simulink library "Model_GridElem_Arc_Fault"  (R2022b)
settings: Solver=VariableStepAuto  StartTime=0.0  StopTime=10.0  RelTol=1e-3
undefined symbols (not defined in the file): DiscIntNeverNeededParam
libraries: powerlib x220, spsVariableResistorLib x3, spsControlledVoltageSourceLib x3, spsGroundLib x1, spsThreePhaseVIMeasurementLib x1
(part 2 of 2)

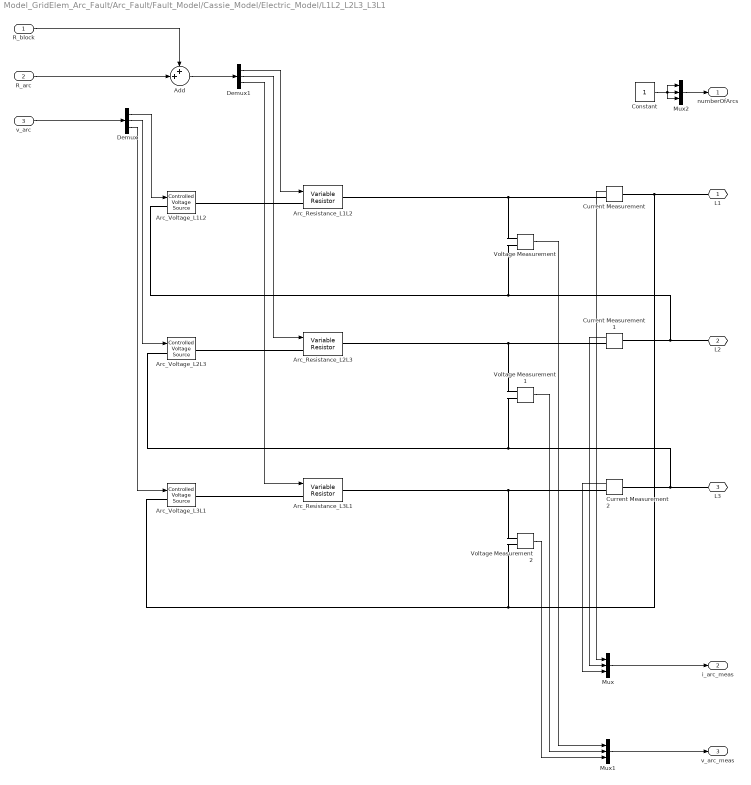
== system Model_GridElem_Arc_Fault/Arc_Fault/Fault_Model/Cassie_Model/Electric_Model/L1L2_L2L3_L3L1 ==
  R_block : Inport
  R_arc : Inport  Port=2
  v_arc : Inport  Port=3
  Add : Sum  Inputs=++|
  Arc_Resistance_L1L2 : powerlib/Elements/Variable Resistor  Rabsmin=1e-6
  Arc_Resistance_L2L3 : powerlib/Elements/Variable Resistor  Rabsmin=1e-6
  Arc_Resistance_L3L1 : powerlib/Elements/Variable Resistor  Rabsmin=1e-6
  Arc_Voltage_L1L2 : powerlib/Electrical Sources/Controlled Voltage Source  Initialize=on  Source_Type=AC  Amplitude=0  Phase=0  Frequency=0  Measurements=None
  Arc_Voltage_L2L3 : powerlib/Electrical Sources/Controlled Voltage Source  Initialize=on  Source_Type=AC  Amplitude=0  Phase=0  Frequency=0  Measurements=None
  Arc_Voltage_L3L1 : powerlib/Electrical Sources/Controlled Voltage Source  Initialize=on  Source_Type=AC  Amplitude=0  Phase=0  Frequency=0  Measurements=None
  Constant : Constant
  Current Measurement : powerlib/Measurements/Current Measurement  PhasorSimulation=off  OutputType=Complex  PSBequivalent=0
  Current Measurement1 : powerlib/Measurements/Current Measurement  PhasorSimulation=off  OutputType=Complex  PSBequivalent=0
  Current Measurement2 : powerlib/Measurements/Current Measurement  PhasorSimulation=off  OutputType=Complex  PSBequivalent=0
  Demux : Demux  Outputs=3
  Demux1 : Demux  Outputs=3
  Mux : Mux  Inputs=3
  Mux1 : Mux  Inputs=3
  Mux2 : Mux  Inputs=3
  Voltage Measurement : powerlib/Measurements/Voltage Measurement  PhasorSimulation=off  OutputType=Complex  PSBequivalent=0
  Voltage Measurement1 : powerlib/Measurements/Voltage Measurement  PhasorSimulation=off  OutputType=Complex  PSBequivalent=0
  Voltage Measurement2 : powerlib/Measurements/Voltage Measurement  PhasorSimulation=off  OutputType=Complex  PSBequivalent=0
  L1 : PMIOPort  Side=Right
  L2 : PMIOPort  Port=2  Side=Right
  L3 : PMIOPort  Port=3  Side=Right
  numberOfArcs : Outport
  i_arc_meas : Outport  Port=2
  v_arc_meas : Outport  Port=3
  wires:
  Constant/1 -> Mux2/2, Mux2/1, Mux2/3
  Mux2/1 -> numberOfArcs/1
  R_arc/1 -> Add/2
  Add/1 -> Demux1/1
  Voltage Measurement2/1 -> Mux1/3
  Voltage Measurement1/1 -> Mux1/2
  Voltage Measurement/1 -> Mux1/1
  Current Measurement2/1 -> Mux/3
  Current Measurement1/1 -> Mux/2
  Current Measurement/1 -> Mux/1
  Mux1/1 -> v_arc_meas/1
  Mux/1 -> i_arc_meas/1
  Demux/2 -> Arc_Voltage_L2L3/1
  Demux1/2 -> Arc_Resistance_L2L3/1
  Demux/3 -> Arc_Voltage_L3L1/1
  Demux1/1 -> Arc_Resistance_L1L2/1
  v_arc/1 -> Demux/1
  Demux/1 -> Arc_Voltage_L1L2/1
  Demux1/3 -> Arc_Resistance_L3L1/1
  R_block/1 -> Add/1
  connections:
  Arc_Resistance_L3L1/RConn1 -- Voltage Measurement2/LConn1 -- Current Measurement2/RConn1
  Arc_Resistance_L2L3/RConn1 -- Voltage Measurement1/LConn1 -- Current Measurement1/RConn1
  Voltage Measurement/LConn1 -- Arc_Resistance_L1L2/RConn1 -- Current Measurement/RConn1
  Current Measurement1/LConn1 -- Voltage Measurement/LConn2 -- Arc_Voltage_L1L2/LConn1 -- L2/RConn1
  L3/RConn1 -- Current Measurement2/LConn1 -- Voltage Measurement1/LConn2 -- Arc_Voltage_L2L3/LConn1
  Current Measurement/LConn1 -- L1/RConn1 -- Voltage Measurement2/LConn2 -- Arc_Voltage_L3L1/LConn1
  Arc_Voltage_L2L3/RConn1 -- Arc_Resistance_L2L3/LConn1
  Arc_Voltage_L3L1/RConn1 -- Arc_Resistance_L3L1/LConn1
  Arc_Voltage_L1L2/RConn1 -- Arc_Resistance_L1L2/LConn1

== system Model_GridElem_Arc_Fault/Arc_Fault/Fault_Model/Mayr_Model/Electric_Model/L1G ==
  R_block : Inport
  R_arc : Inport  Port=2
  v_arc : Inport  Port=3
  Add : Sum  Inputs=++|
  Arc_Resistance_L1G : powerlib/Elements/Variable Resistor  Rabsmin=1e-6
  Arc_Voltage_L1G : powerlib/Electrical Sources/Controlled Voltage Source  Initialize=on  Source_Type=AC  Amplitude=0  Phase=0  Frequency=0  Measurements=None
  Constant : Constant
  Current Measurement : powerlib/Measurements/Current Measurement  PhasorSimulation=off  OutputType=Complex  PSBequivalent=0
  Ground{,1..3} (4 alike) : powerlib/Elements/Ground  LConnTagsString=a
  Terminator : Terminator
  Terminator1 : Terminator
  Voltage Measurement : powerlib/Measurements/Voltage Measurement  PhasorSimulation=off  OutputType=Complex  PSBequivalent=0
  Voltage Measurement1 : powerlib/Measurements/Voltage Measurement  PhasorSimulation=off  OutputType=Complex  PSBequivalent=0
  Voltage Measurement2 : powerlib/Measurements/Voltage Measurement  PhasorSimulation=off  OutputType=Complex  PSBequivalent=0
  L1 : PMIOPort  Side=Right
  L2 : PMIOPort  Port=2  Side=Right
  L3 : PMIOPort  Port=3  Side=Right
  numberOfArcs : Outport
  i_arc_meas : Outport  Port=2
  v_arc_meas : Outport  Port=3
  wires:
  Constant/1 -> numberOfArcs/1
  Add/1 -> Arc_Resistance_L1G/1
  R_block/1 -> Add/1
  R_arc/1 -> Add/2
  Voltage Measurement1/1 -> Terminator1/1
  Current Measurement/1 -> i_arc_meas/1
  v_arc/1 -> Arc_Voltage_L1G/1
  Voltage Measurement2/1 -> Terminator/1
  Voltage Measurement/1 -> v_arc_meas/1
  connections:
  Voltage Measurement1/LConn2 -- Ground2/LConn1
  Voltage Measurement1/LConn1 -- L2/RConn1
  Arc_Voltage_L1G/RConn1 -- Arc_Resistance_L1G/LConn1
  Voltage Measurement2/LConn2 -- Ground3/LConn1
  Ground1/LConn1 -- Voltage Measurement/LConn2
  Voltage Measurement2/LConn1 -- L3/RConn1
  Current Measurement/LConn1 -- L1/RConn1
  Ground/LConn1 -- Arc_Voltage_L1G/LConn1
  Voltage Measurement/LConn1 -- Arc_Resistance_L1G/RConn1 -- Current Measurement/RConn1

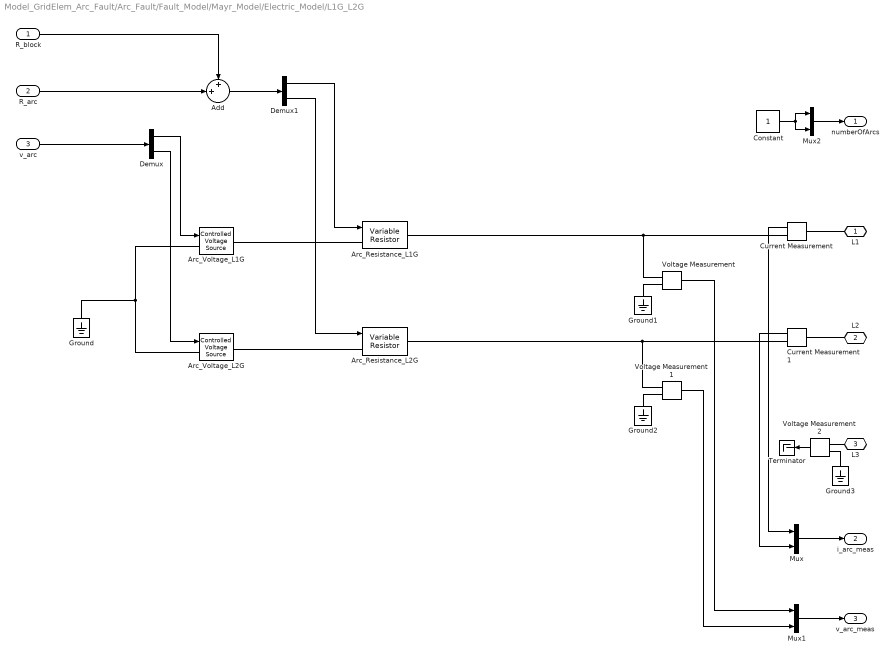
== system Model_GridElem_Arc_Fault/Arc_Fault/Fault_Model/Mayr_Model/Electric_Model/L1G_L2G ==
  R_block : Inport
  R_arc : Inport  Port=2
  v_arc : Inport  Port=3
  Add : Sum  Inputs=++|
  Arc_Resistance_L1G : powerlib/Elements/Variable Resistor  Rabsmin=1e-6
  Arc_Resistance_L2G : powerlib/Elements/Variable Resistor  Rabsmin=1e-6
  Arc_Voltage_L1G : powerlib/Electrical Sources/Controlled Voltage Source  Initialize=on  Source_Type=AC  Amplitude=0  Phase=0  Frequency=0  Measurements=None
  Arc_Voltage_L2G : powerlib/Electrical Sources/Controlled Voltage Source  Initialize=on  Source_Type=AC  Amplitude=0  Phase=0  Frequency=0  Measurements=None
  Constant : Constant
  Current Measurement : powerlib/Measurements/Current Measurement  PhasorSimulation=off  OutputType=Complex  PSBequivalent=0
  Current Measurement1 : powerlib/Measurements/Current Measurement  PhasorSimulation=off  OutputType=Complex  PSBequivalent=0
  Demux : Demux  Outputs=2
  Demux1 : Demux  Outputs=2
  Ground{,1..3} (4 alike) : powerlib/Elements/Ground  LConnTagsString=a
  Mux : Mux  Inputs=2
  Mux1 : Mux  Inputs=2
  Mux2 : Mux  Inputs=2
  Terminator : Terminator
  Voltage Measurement : powerlib/Measurements/Voltage Measurement  PhasorSimulation=off  OutputType=Complex  PSBequivalent=0
  Voltage Measurement1 : powerlib/Measurements/Voltage Measurement  PhasorSimulation=off  OutputType=Complex  PSBequivalent=0
  Voltage Measurement2 : powerlib/Measurements/Voltage Measurement  PhasorSimulation=off  OutputType=Complex  PSBequivalent=0
  L1 : PMIOPort  Side=Right
  L2 : PMIOPort  Port=2  Side=Right
  L3 : PMIOPort  Port=3  Side=Right
  numberOfArcs : Outport
  i_arc_meas : Outport  Port=2
  v_arc_meas : Outport  Port=3
  wires:
  Constant/1 -> Mux2/1, Mux2/2
  Mux2/1 -> numberOfArcs/1
  R_block/1 -> Add/1
  Add/1 -> Demux1/1
  R_arc/1 -> Add/2
  Voltage Measurement2/1 -> Terminator/1
  Voltage Measurement1/1 -> Mux1/2
  Voltage Measurement/1 -> Mux1/1
  Current Measurement1/1 -> Mux/2
  Current Measurement/1 -> Mux/1
  Mux1/1 -> v_arc_meas/1
  Mux/1 -> i_arc_meas/1
  Demux/2 -> Arc_Voltage_L2G/1
  Demux1/2 -> Arc_Resistance_L2G/1
  Demux1/1 -> Arc_Resistance_L1G/1
  v_arc/1 -> Demux/1
  Demux/1 -> Arc_Voltage_L1G/1
  connections:
  Voltage Measurement2/LConn2 -- Ground3/LConn1
  Ground2/LConn1 -- Voltage Measurement1/LConn2
  Ground1/LConn1 -- Voltage Measurement/LConn2
  Current Measurement1/LConn1 -- L2/RConn1
  Voltage Measurement1/LConn1 -- Arc_Resistance_L2G/RConn1 -- Current Measurement1/RConn1
  Current Measurement/LConn1 -- L1/RConn1
  Voltage Measurement/LConn1 -- Arc_Resistance_L1G/RConn1 -- Current Measurement/RConn1
  Arc_Voltage_L1G/RConn1 -- Arc_Resistance_L1G/LConn1
  Arc_Voltage_L2G/RConn1 -- Arc_Resistance_L2G/LConn1
  Voltage Measurement2/LConn1 -- L3/RConn1
  Arc_Voltage_L1G/LConn1 -- Arc_Voltage_L2G/LConn1 -- Ground/LConn1

== system Model_GridElem_Arc_Fault/Arc_Fault/Fault_Model/Mayr_Model/Electric_Model/L1G_L2G_L3G ==
  R_block : Inport
  R_arc : Inport  Port=2
  v_arc : Inport  Port=3
  Add : Sum  Inputs=++|
  Arc_Resistance_L1G : powerlib/Elements/Variable Resistor  Rabsmin=1e-6
  Arc_Resistance_L2G : powerlib/Elements/Variable Resistor  Rabsmin=1e-6
  Arc_Resistance_L3G : powerlib/Elements/Variable Resistor  Rabsmin=1e-6
  Arc_Voltage_L1G : powerlib/Electrical Sources/Controlled Voltage Source  Initialize=on  Source_Type=AC  Amplitude=0  Phase=0  Frequency=0  Measurements=None
  Arc_Voltage_L2G : powerlib/Electrical Sources/Controlled Voltage Source  Initialize=on  Source_Type=AC  Amplitude=0  Phase=0  Frequency=0  Measurements=None
  Arc_Voltage_L3G : powerlib/Electrical Sources/Controlled Voltage Source  Initialize=on  Source_Type=AC  Amplitude=0  Phase=0  Frequency=0  Measurements=None
  Constant : Constant
  Demux : Demux  Outputs=3
  Demux1 : Demux  Outputs=3
  Ground : powerlib/Elements/Ground  LConnTagsString=a
  Mux : Mux  Inputs=3
  Three-Phase V-I Measurement : powerlib/Measurements/Three-Phase V-I Measurement  VoltageMeasurement=phase-to-ground  SetLabelV=off  LabelV=Vabc  Vpu=off  VpuLL=off  CurrentMeasurement=yes  SetLabelI=off  LabelI=Iabc  Ipu=off  Pbase=100e6  Vbase=500e3  OutputType=Complex  PhasorSimulation=off  PSBequivalent=0
  L1 : PMIOPort  Side=Right
  L2 : PMIOPort  Port=2  Side=Right
  L3 : PMIOPort  Port=3  Side=Right
  numberOfArcs : Outport
  i_arc_meas : Outport  Port=2
  v_arc_meas : Outport  Port=3
  wires:
  Constant/1 -> Mux/2, Mux/1, Mux/3
  Mux/1 -> numberOfArcs/1
  R_block/1 -> Add/1
  Add/1 -> Demux1/1
  R_arc/1 -> Add/2
  Demux1/1 -> Arc_Resistance_L1G/1
  Demux1/2 -> Arc_Resistance_L2G/1
  Demux1/3 -> Arc_Resistance_L3G/1
  Demux/1 -> Arc_Voltage_L1G/1
  Demux/2 -> Arc_Voltage_L2G/1
  Demux/3 -> Arc_Voltage_L3G/1
  Three-Phase V-I Measurement/1 -> v_arc_meas/1
  Three-Phase V-I Measurement/2 -> i_arc_meas/1
  v_arc/1 -> Demux/1
  connections:
  Three-Phase V-I Measurement/LConn3 -- L3/RConn1
  Three-Phase V-I Measurement/LConn2 -- L2/RConn1
  Three-Phase V-I Measurement/LConn1 -- L1/RConn1
  Arc_Resistance_L3G/RConn1 -- Three-Phase V-I Measurement/RConn3
  Arc_Resistance_L1G/RConn1 -- Three-Phase V-I Measurement/RConn1
  Ground/LConn1 -- Arc_Voltage_L3G/LConn1 -- Arc_Voltage_L2G/LConn1 -- Arc_Voltage_L1G/LConn1
  Arc_Voltage_L3G/RConn1 -- Arc_Resistance_L3G/LConn1
  Arc_Voltage_L2G/RConn1 -- Arc_Resistance_L2G/LConn1
  Arc_Voltage_L1G/RConn1 -- Arc_Resistance_L1G/LConn1
  Three-Phase V-I Measurement/RConn2 -- Arc_Resistance_L2G/RConn1

== system Model_GridElem_Arc_Fault/Arc_Fault/Fault_Model/Mayr_Model/Electric_Model/L1L2 ==
  R_block : Inport
  R_arc : Inport  Port=2
  v_arc : Inport  Port=3
  Add : Sum  Inputs=++|
  Arc_Resistance_L1L2 : powerlib/Elements/Variable Resistor  Rabsmin=1e-6
  Arc_Voltage_L1L2 : powerlib/Electrical Sources/Controlled Voltage Source  Initialize=on  Source_Type=AC  Amplitude=0  Phase=0  Frequency=0  Measurements=None
  Constant : Constant
  Current Measurement : powerlib/Measurements/Current Measurement  PhasorSimulation=off  OutputType=Complex  PSBequivalent=0
  Ground : powerlib/Elements/Ground  LConnTagsString=a
  Terminator : Terminator
  Voltage Measurement : powerlib/Measurements/Voltage Measurement  PhasorSimulation=off  OutputType=Complex  PSBequivalent=0
  Voltage Measurement1 : powerlib/Measurements/Voltage Measurement  PhasorSimulation=off  OutputType=Complex  PSBequivalent=0
  L1 : PMIOPort  Side=Right
  L2 : PMIOPort  Port=2  Side=Right
  L3 : PMIOPort  Port=3  Side=Right
  numberOfArcs : Outport
  i_arc_meas : Outport  Port=2
  v_arc_meas : Outport  Port=3
  wires:
  Constant/1 -> numberOfArcs/1
  R_block/1 -> Add/1
  Add/1 -> Arc_Resistance_L1L2/1
  R_arc/1 -> Add/2
  Voltage Measurement1/1 -> Terminator/1
  v_arc/1 -> Arc_Voltage_L1L2/1
  Voltage Measurement/1 -> v_arc_meas/1
  Current Measurement/1 -> i_arc_meas/1
  connections:
  Voltage Measurement1/LConn2 -- Ground/LConn1
  Voltage Measurement1/LConn1 -- L3/RConn1
  Arc_Voltage_L1L2/RConn1 -- Arc_Resistance_L1L2/LConn1
  Current Measurement/LConn1 -- L1/RConn1
  L2/RConn1 -- Arc_Voltage_L1L2/LConn1 -- Voltage Measurement/LConn2
  Voltage Measurement/LConn1 -- Arc_Resistance_L1L2/RConn1 -- Current Measurement/RConn1

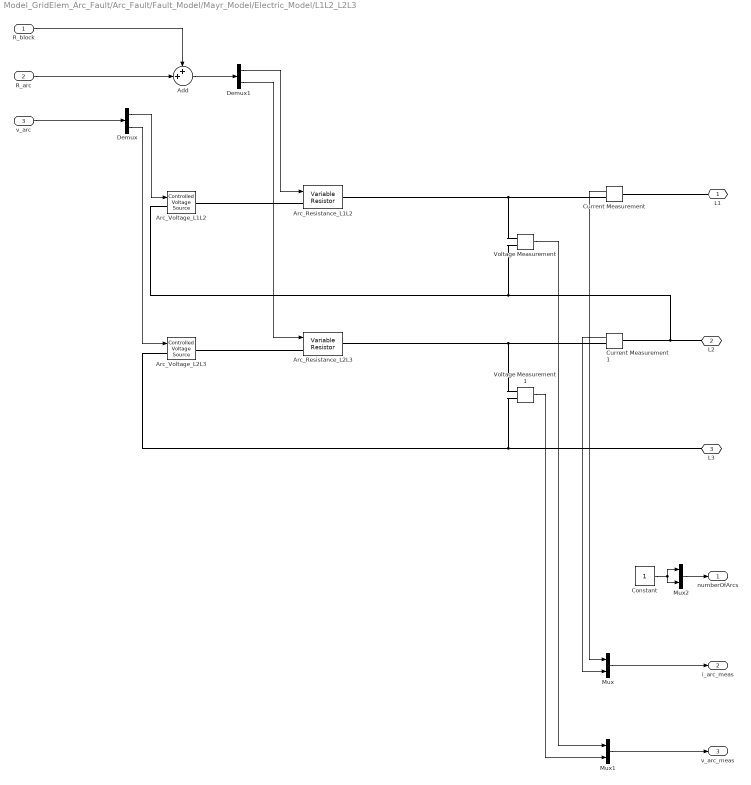
== system Model_GridElem_Arc_Fault/Arc_Fault/Fault_Model/Mayr_Model/Electric_Model/L1L2_L2L3 ==
  R_block : Inport
  R_arc : Inport  Port=2
  v_arc : Inport  Port=3
  Add : Sum  Inputs=++|
  Arc_Resistance_L1L2 : powerlib/Elements/Variable Resistor  Rabsmin=1e-6
  Arc_Resistance_L2L3 : powerlib/Elements/Variable Resistor  Rabsmin=1e-6
  Arc_Voltage_L1L2 : powerlib/Electrical Sources/Controlled Voltage Source  Initialize=on  Source_Type=AC  Amplitude=0  Phase=0  Frequency=0  Measurements=None
  Arc_Voltage_L2L3 : powerlib/Electrical Sources/Controlled Voltage Source  Initialize=on  Source_Type=AC  Amplitude=0  Phase=0  Frequency=0  Measurements=None
  Constant : Constant
  Current Measurement : powerlib/Measurements/Current Measurement  PhasorSimulation=off  OutputType=Complex  PSBequivalent=0
  Current Measurement1 : powerlib/Measurements/Current Measurement  PhasorSimulation=off  OutputType=Complex  PSBequivalent=0
  Demux : Demux  Outputs=2
  Demux1 : Demux  Outputs=2
  Mux : Mux  Inputs=2
  Mux1 : Mux  Inputs=2
  Mux2 : Mux  Inputs=2
  Voltage Measurement : powerlib/Measurements/Voltage Measurement  PhasorSimulation=off  OutputType=Complex  PSBequivalent=0
  Voltage Measurement1 : powerlib/Measurements/Voltage Measurement  PhasorSimulation=off  OutputType=Complex  PSBequivalent=0
  L1 : PMIOPort  Side=Right
  L2 : PMIOPort  Port=2  Side=Right
  L3 : PMIOPort  Port=3  Side=Right
  numberOfArcs : Outport
  i_arc_meas : Outport  Port=2
  v_arc_meas : Outport  Port=3
  wires:
  Constant/1 -> Mux2/1, Mux2/2
  Mux2/1 -> numberOfArcs/1
  R_block/1 -> Add/1
  R_arc/1 -> Add/2
  Add/1 -> Demux1/1
  Demux1/2 -> Arc_Resistance_L2L3/1
  Voltage Measurement1/1 -> Mux1/2
  Voltage Measurement/1 -> Mux1/1
  Demux/2 -> Arc_Voltage_L2L3/1
  Demux1/1 -> Arc_Resistance_L1L2/1
  Mux1/1 -> v_arc_meas/1
  Demux/1 -> Arc_Voltage_L1L2/1
  v_arc/1 -> Demux/1
  Current Measurement1/1 -> Mux/2
  Mux/1 -> i_arc_meas/1
  Current Measurement/1 -> Mux/1
  connections:
  Arc_Voltage_L1L2/RConn1 -- Arc_Resistance_L1L2/LConn1
  Arc_Voltage_L2L3/RConn1 -- Arc_Resistance_L2L3/LConn1
  Voltage Measurement1/LConn1 -- Arc_Resistance_L2L3/RConn1 -- Current Measurement1/RConn1
  Arc_Voltage_L1L2/LConn1 -- L2/RConn1 -- Current Measurement1/LConn1 -- Voltage Measurement/LConn2
  L3/RConn1 -- Arc_Voltage_L2L3/LConn1 -- Voltage Measurement1/LConn2
  Voltage Measurement/LConn1 -- Arc_Resistance_L1L2/RConn1 -- Current Measurement/RConn1
  Current Measurement/LConn1 -- L1/RConn1

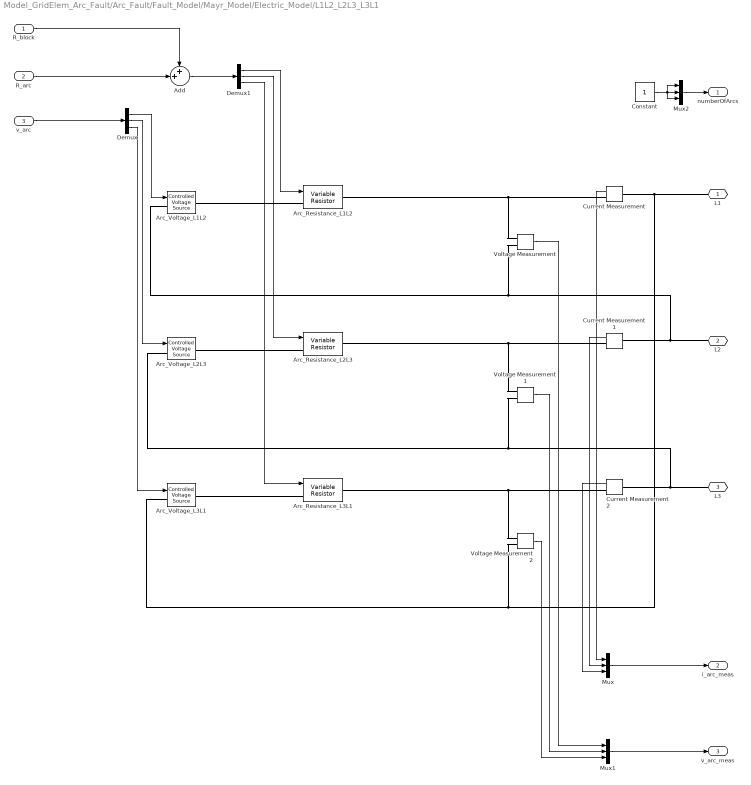
== system Model_GridElem_Arc_Fault/Arc_Fault/Fault_Model/Mayr_Model/Electric_Model/L1L2_L2L3_L3L1 ==
  R_block : Inport
  R_arc : Inport  Port=2
  v_arc : Inport  Port=3
  Add : Sum  Inputs=++|
  Arc_Resistance_L1L2 : powerlib/Elements/Variable Resistor  Rabsmin=1e-6
  Arc_Resistance_L2L3 : powerlib/Elements/Variable Resistor  Rabsmin=1e-6
  Arc_Resistance_L3L1 : powerlib/Elements/Variable Resistor  Rabsmin=1e-6
  Arc_Voltage_L1L2 : powerlib/Electrical Sources/Controlled Voltage Source  Initialize=on  Source_Type=AC  Amplitude=0  Phase=0  Frequency=0  Measurements=None
  Arc_Voltage_L2L3 : powerlib/Electrical Sources/Controlled Voltage Source  Initialize=on  Source_Type=AC  Amplitude=0  Phase=0  Frequency=0  Measurements=None
  Arc_Voltage_L3L1 : powerlib/Electrical Sources/Controlled Voltage Source  Initialize=on  Source_Type=AC  Amplitude=0  Phase=0  Frequency=0  Measurements=None
  Constant : Constant
  Current Measurement : powerlib/Measurements/Current Measurement  PhasorSimulation=off  OutputType=Complex  PSBequivalent=0
  Current Measurement1 : powerlib/Measurements/Current Measurement  PhasorSimulation=off  OutputType=Complex  PSBequivalent=0
  Current Measurement2 : powerlib/Measurements/Current Measurement  PhasorSimulation=off  OutputType=Complex  PSBequivalent=0
  Demux : Demux  Outputs=3
  Demux1 : Demux  Outputs=3
  Mux : Mux  Inputs=3
  Mux1 : Mux  Inputs=3
  Mux2 : Mux  Inputs=3
  Voltage Measurement : powerlib/Measurements/Voltage Measurement  PhasorSimulation=off  OutputType=Complex  PSBequivalent=0
  Voltage Measurement1 : powerlib/Measurements/Voltage Measurement  PhasorSimulation=off  OutputType=Complex  PSBequivalent=0
  Voltage Measurement2 : powerlib/Measurements/Voltage Measurement  PhasorSimulation=off  OutputType=Complex  PSBequivalent=0
  L1 : PMIOPort  Side=Right
  L2 : PMIOPort  Port=2  Side=Right
  L3 : PMIOPort  Port=3  Side=Right
  numberOfArcs : Outport
  i_arc_meas : Outport  Port=2
  v_arc_meas : Outport  Port=3
  wires:
  Constant/1 -> Mux2/2, Mux2/1, Mux2/3
  Mux2/1 -> numberOfArcs/1
  R_arc/1 -> Add/2
  Add/1 -> Demux1/1
  Voltage Measurement2/1 -> Mux1/3
  Voltage Measurement1/1 -> Mux1/2
  Voltage Measurement/1 -> Mux1/1
  Current Measurement2/1 -> Mux/3
  Current Measurement1/1 -> Mux/2
  Current Measurement/1 -> Mux/1
  Mux1/1 -> v_arc_meas/1
  Mux/1 -> i_arc_meas/1
  Demux/2 -> Arc_Voltage_L2L3/1
  Demux1/2 -> Arc_Resistance_L2L3/1
  Demux/3 -> Arc_Voltage_L3L1/1
  Demux1/1 -> Arc_Resistance_L1L2/1
  v_arc/1 -> Demux/1
  Demux/1 -> Arc_Voltage_L1L2/1
  Demux1/3 -> Arc_Resistance_L3L1/1
  R_block/1 -> Add/1
  connections:
  Arc_Resistance_L3L1/RConn1 -- Voltage Measurement2/LConn1 -- Current Measurement2/RConn1
  Arc_Resistance_L2L3/RConn1 -- Voltage Measurement1/LConn1 -- Current Measurement1/RConn1
  Voltage Measurement/LConn1 -- Arc_Resistance_L1L2/RConn1 -- Current Measurement/RConn1
  Current Measurement1/LConn1 -- Voltage Measurement/LConn2 -- Arc_Voltage_L1L2/LConn1 -- L2/RConn1
  L3/RConn1 -- Current Measurement2/LConn1 -- Voltage Measurement1/LConn2 -- Arc_Voltage_L2L3/LConn1
  Current Measurement/LConn1 -- L1/RConn1 -- Voltage Measurement2/LConn2 -- Arc_Voltage_L3L1/LConn1
  Arc_Voltage_L2L3/RConn1 -- Arc_Resistance_L2L3/LConn1
  Arc_Voltage_L3L1/RConn1 -- Arc_Resistance_L3L1/LConn1
  Arc_Voltage_L1L2/RConn1 -- Arc_Resistance_L1L2/LConn1

== system Model_GridElem_Arc_Fault/Arc_Fault/Fault_Model/Mayr_Model/Mayr_Arc_Model/Arc_Equations ==
  enable : Inport
  numberOfArcs : Inport  Port=2
  i_abc : Inport  Port=3
  Enable : EnablePort
  1/P : Gain  Gain=1/Mayr_P_0
  1/T : Gain  Gain=1/Mayr_T
  Add : Sum  Inputs=|+-
  Constant : Constant  Value=(Mayr_G_max-Mayr_G_min)/2
  Discrete-Time Integrator : DiscreteIntegrator  ExternalReset=rising  InitialConditionSource=external  SampleTime=-1  LimitOutput=on  UpperSaturationLimit=Mayr_G_max  LowerSaturationLimit=Mayr_G_min  IgnoreLimit=on  ICPrevOutput=DiscIntNeverNeededParam  ICPrevScaledInput=DiscIntNeverNeededParam
  Divide : Product  Inputs=**
  Math Function : Math  Operator=square
  Math Function1 : Math  Operator=reciprocal
  R_arc : Outport
  wires:
  Math Function1/1 -> R_arc/1
  i_abc/1 -> Math Function/1
  Math Function/1 -> 1/P/1
  1/P/1 -> Add/1
  Add/1 -> 1/T/1
  1/T/1 -> Discrete-Time Integrator/1
  enable/1 -> Discrete-Time Integrator/2
  Discrete-Time Integrator/1 -> Math Function1/1, Add/2
  Divide/1 -> Discrete-Time Integrator/3
  Constant/1 -> Divide/1
  numberOfArcs/1 -> Divide/2

== system Model_GridElem_Arc_Fault/Arc_Fault/Fault_Model/Resistor/Electric_Model/L1G ==
  R_block : Inport
  R_arc : Inport  Port=2
  v_arc : Inport  Port=3
  Add : Sum  Inputs=++|
  Arc_Resistance_L1G : powerlib/Elements/Variable Resistor  Rabsmin=1e-6
  Arc_Voltage_L1G : powerlib/Electrical Sources/Controlled Voltage Source  Initialize=on  Source_Type=AC  Amplitude=0  Phase=0  Frequency=0  Measurements=None
  Constant : Constant
  Current Measurement : powerlib/Measurements/Current Measurement  PhasorSimulation=off  OutputType=Complex  PSBequivalent=0
  Ground{,1..3} (4 alike) : powerlib/Elements/Ground  LConnTagsString=a
  Terminator : Terminator
  Terminator1 : Terminator
  Voltage Measurement : powerlib/Measurements/Voltage Measurement  PhasorSimulation=off  OutputType=Complex  PSBequivalent=0
  Voltage Measurement1 : powerlib/Measurements/Voltage Measurement  PhasorSimulation=off  OutputType=Complex  PSBequivalent=0
  Voltage Measurement2 : powerlib/Measurements/Voltage Measurement  PhasorSimulation=off  OutputType=Complex  PSBequivalent=0
  L1 : PMIOPort  Side=Right
  L2 : PMIOPort  Port=2  Side=Right
  L3 : PMIOPort  Port=3  Side=Right
  numberOfArcs : Outport
  i_arc_meas : Outport  Port=2
  v_arc_meas : Outport  Port=3
  wires:
  Voltage Measurement/1 -> v_arc_meas/1
  Voltage Measurement2/1 -> Terminator/1
  v_arc/1 -> Arc_Voltage_L1G/1
  Current Measurement/1 -> i_arc_meas/1
  Voltage Measurement1/1 -> Terminator1/1
  R_arc/1 -> Add/2
  R_block/1 -> Add/1
  Add/1 -> Arc_Resistance_L1G/1
  Constant/1 -> numberOfArcs/1
  connections:
  Current Measurement/RConn1 -- Arc_Resistance_L1G/RConn1 -- Voltage Measurement/LConn1
  Ground/LConn1 -- Arc_Voltage_L1G/LConn1
  Current Measurement/LConn1 -- L1/RConn1
  Voltage Measurement2/LConn1 -- L3/RConn1
  Ground1/LConn1 -- Voltage Measurement/LConn2
  Voltage Measurement2/LConn2 -- Ground3/LConn1
  Arc_Voltage_L1G/RConn1 -- Arc_Resistance_L1G/LConn1
  Voltage Measurement1/LConn1 -- L2/RConn1
  Voltage Measurement1/LConn2 -- Ground2/LConn1

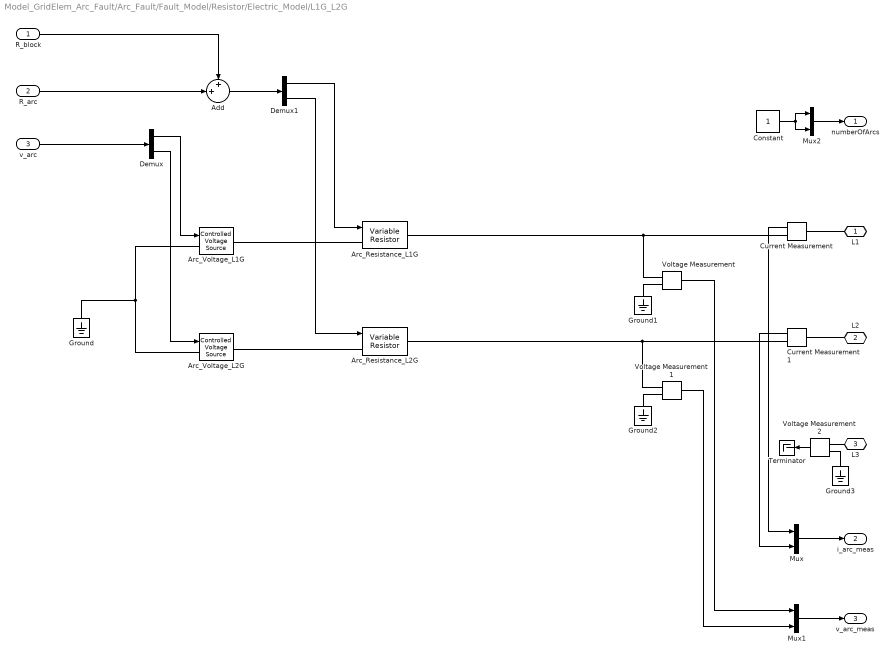
== system Model_GridElem_Arc_Fault/Arc_Fault/Fault_Model/Resistor/Electric_Model/L1G_L2G ==
  R_block : Inport
  R_arc : Inport  Port=2
  v_arc : Inport  Port=3
  Add : Sum  Inputs=++|
  Arc_Resistance_L1G : powerlib/Elements/Variable Resistor  Rabsmin=1e-6
  Arc_Resistance_L2G : powerlib/Elements/Variable Resistor  Rabsmin=1e-6
  Arc_Voltage_L1G : powerlib/Electrical Sources/Controlled Voltage Source  Initialize=on  Source_Type=AC  Amplitude=0  Phase=0  Frequency=0  Measurements=None
  Arc_Voltage_L2G : powerlib/Electrical Sources/Controlled Voltage Source  Initialize=on  Source_Type=AC  Amplitude=0  Phase=0  Frequency=0  Measurements=None
  Constant : Constant
  Current Measurement : powerlib/Measurements/Current Measurement  PhasorSimulation=off  OutputType=Complex  PSBequivalent=0
  Current Measurement1 : powerlib/Measurements/Current Measurement  PhasorSimulation=off  OutputType=Complex  PSBequivalent=0
  Demux : Demux  Outputs=2
  Demux1 : Demux  Outputs=2
  Ground{,1..3} (4 alike) : powerlib/Elements/Ground  LConnTagsString=a
  Mux : Mux  Inputs=2
  Mux1 : Mux  Inputs=2
  Mux2 : Mux  Inputs=2
  Terminator : Terminator
  Voltage Measurement : powerlib/Measurements/Voltage Measurement  PhasorSimulation=off  OutputType=Complex  PSBequivalent=0
  Voltage Measurement1 : powerlib/Measurements/Voltage Measurement  PhasorSimulation=off  OutputType=Complex  PSBequivalent=0
  Voltage Measurement2 : powerlib/Measurements/Voltage Measurement  PhasorSimulation=off  OutputType=Complex  PSBequivalent=0
  L1 : PMIOPort  Side=Right
  L2 : PMIOPort  Port=2  Side=Right
  L3 : PMIOPort  Port=3  Side=Right
  numberOfArcs : Outport
  i_arc_meas : Outport  Port=2
  v_arc_meas : Outport  Port=3
  wires:
  Demux/1 -> Arc_Voltage_L1G/1
  v_arc/1 -> Demux/1
  Demux1/1 -> Arc_Resistance_L1G/1
  Demux1/2 -> Arc_Resistance_L2G/1
  Demux/2 -> Arc_Voltage_L2G/1
  Mux/1 -> i_arc_meas/1
  Mux1/1 -> v_arc_meas/1
  Current Measurement/1 -> Mux/1
  Current Measurement1/1 -> Mux/2
  Voltage Measurement/1 -> Mux1/1
  Voltage Measurement1/1 -> Mux1/2
  Voltage Measurement2/1 -> Terminator/1
  R_arc/1 -> Add/2
  Add/1 -> Demux1/1
  R_block/1 -> Add/1
  Mux2/1 -> numberOfArcs/1
  Constant/1 -> Mux2/2, Mux2/1
  connections:
  Ground/LConn1 -- Arc_Voltage_L2G/LConn1 -- Arc_Voltage_L1G/LConn1
  Voltage Measurement2/LConn1 -- L3/RConn1
  Arc_Voltage_L2G/RConn1 -- Arc_Resistance_L2G/LConn1
  Arc_Voltage_L1G/RConn1 -- Arc_Resistance_L1G/LConn1
  Current Measurement/RConn1 -- Arc_Resistance_L1G/RConn1 -- Voltage Measurement/LConn1
  Current Measurement/LConn1 -- L1/RConn1
  Current Measurement1/RConn1 -- Arc_Resistance_L2G/RConn1 -- Voltage Measurement1/LConn1
  Current Measurement1/LConn1 -- L2/RConn1
  Ground1/LConn1 -- Voltage Measurement/LConn2
  Ground2/LConn1 -- Voltage Measurement1/LConn2
  Voltage Measurement2/LConn2 -- Ground3/LConn1

== system Model_GridElem_Arc_Fault/Arc_Fault/Fault_Model/Resistor/Electric_Model/L1G_L2G_L3G ==
  R_block : Inport
  R_arc : Inport  Port=2
  v_arc : Inport  Port=3
  Add : Sum  Inputs=++|
  Arc_Resistance_L1G : spsVariableResistorLib/Variable Resistor  Rabsmin=1e-6
  Arc_Resistance_L2G : spsVariableResistorLib/Variable Resistor  Rabsmin=1e-6
  Arc_Resistance_L3G : spsVariableResistorLib/Variable Resistor  Rabsmin=1e-6
  Arc_Voltage_L1G : spsControlledVoltageSourceLib/Controlled Voltage Source  Initialize=on  Source_Type=AC  Amplitude=0  Phase=0  Frequency=0  Measurements=None
  Arc_Voltage_L2G : spsControlledVoltageSourceLib/Controlled Voltage Source  Initialize=on  Source_Type=AC  Amplitude=0  Phase=0  Frequency=0  Measurements=None
  Arc_Voltage_L3G : spsControlledVoltageSourceLib/Controlled Voltage Source  Initialize=on  Source_Type=AC  Amplitude=0  Phase=0  Frequency=0  Measurements=None
  Constant : Constant
  Demux : Demux  Outputs=3
  Demux1 : Demux  Outputs=3
  Ground : spsGroundLib/Ground  LConnTagsString=a
  Mux : Mux  Inputs=3
  Three-Phase V-I Measurement : spsThreePhaseVIMeasurementLib/Three-Phase V-I Measurement  VoltageMeasurement=phase-to-ground  SetLabelV=off  LabelV=Vabc  Vpu=off  VpuLL=off  CurrentMeasurement=yes  SetLabelI=off  LabelI=Iabc  Ipu=off  Pbase=100e6  Vbase=500e3  OutputType=Complex  PhasorSimulation=off  PSBequivalent=0
  L1 : PMIOPort  Side=Right
  L2 : PMIOPort  Port=2  Side=Right
  L3 : PMIOPort  Port=3  Side=Right
  numberOfArcs : Outport
  i_arc_meas : Outport  Port=2
  v_arc_meas : Outport  Port=3
  wires:
  v_arc/1 -> Demux/1
  Three-Phase V-I Measurement/2 -> i_arc_meas/1
  Three-Phase V-I Measurement/1 -> v_arc_meas/1
  Demux/3 -> Arc_Voltage_L3G/1
  Demux/2 -> Arc_Voltage_L2G/1
  Demux/1 -> Arc_Voltage_L1G/1
  Demux1/3 -> Arc_Resistance_L3G/1
  Demux1/2 -> Arc_Resistance_L2G/1
  Demux1/1 -> Arc_Resistance_L1G/1
  R_arc/1 -> Add/2
  Add/1 -> Demux1/1
  R_block/1 -> Add/1
  Mux/1 -> numberOfArcs/1
  Constant/1 -> Mux/3, Mux/1, Mux/2
  connections:
  Three-Phase V-I Measurement/RConn2 -- Arc_Resistance_L2G/RConn1
  Arc_Voltage_L1G/RConn1 -- Arc_Resistance_L1G/LConn1
  Arc_Voltage_L2G/RConn1 -- Arc_Resistance_L2G/LConn1
  Arc_Voltage_L3G/RConn1 -- Arc_Resistance_L3G/LConn1
  Arc_Voltage_L1G/LConn1 -- Arc_Voltage_L2G/LConn1 -- Arc_Voltage_L3G/LConn1 -- Ground/LConn1
  Arc_Resistance_L1G/RConn1 -- Three-Phase V-I Measurement/RConn1
  Arc_Resistance_L3G/RConn1 -- Three-Phase V-I Measurement/RConn3
  Three-Phase V-I Measurement/LConn1 -- L1/RConn1
  Three-Phase V-I Measurement/LConn2 -- L2/RConn1
  Three-Phase V-I Measurement/LConn3 -- L3/RConn1

== system Model_GridElem_Arc_Fault/Arc_Fault/Fault_Model/Resistor/Electric_Model/L1L2 ==
  R_block : Inport
  R_arc : Inport  Port=2
  v_arc : Inport  Port=3
  Add : Sum  Inputs=++|
  Arc_Resistance_L1L2 : powerlib/Elements/Variable Resistor  Rabsmin=1e-6
  Arc_Voltage_L1L2 : powerlib/Electrical Sources/Controlled Voltage Source  Initialize=on  Source_Type=AC  Amplitude=0  Phase=0  Frequency=0  Measurements=None
  Constant : Constant
  Current Measurement : powerlib/Measurements/Current Measurement  PhasorSimulation=off  OutputType=Complex  PSBequivalent=0
  Ground : powerlib/Elements/Ground  LConnTagsString=a
  Terminator : Terminator
  Voltage Measurement : powerlib/Measurements/Voltage Measurement  PhasorSimulation=off  OutputType=Complex  PSBequivalent=0
  Voltage Measurement1 : powerlib/Measurements/Voltage Measurement  PhasorSimulation=off  OutputType=Complex  PSBequivalent=0
  L1 : PMIOPort  Side=Right
  L2 : PMIOPort  Port=2  Side=Right
  L3 : PMIOPort  Port=3  Side=Right
  numberOfArcs : Outport
  i_arc_meas : Outport  Port=2
  v_arc_meas : Outport  Port=3
  wires:
  Current Measurement/1 -> i_arc_meas/1
  Voltage Measurement/1 -> v_arc_meas/1
  v_arc/1 -> Arc_Voltage_L1L2/1
  Voltage Measurement1/1 -> Terminator/1
  R_arc/1 -> Add/2
  Add/1 -> Arc_Resistance_L1L2/1
  R_block/1 -> Add/1
  Constant/1 -> numberOfArcs/1
  connections:
  Current Measurement/RConn1 -- Arc_Resistance_L1L2/RConn1 -- Voltage Measurement/LConn1
  Voltage Measurement/LConn2 -- Arc_Voltage_L1L2/LConn1 -- L2/RConn1
  Current Measurement/LConn1 -- L1/RConn1
  Arc_Voltage_L1L2/RConn1 -- Arc_Resistance_L1L2/LConn1
  Voltage Measurement1/LConn1 -- L3/RConn1
  Voltage Measurement1/LConn2 -- Ground/LConn1

== system Model_GridElem_Arc_Fault/Arc_Fault/Fault_Model/Resistor/Electric_Model/L1L2_L2L3 ==
  R_block : Inport
  R_arc : Inport  Port=2
  v_arc : Inport  Port=3
  Add : Sum  Inputs=++|
  Arc_Resistance_L1L2 : powerlib/Elements/Variable Resistor  Rabsmin=1e-6
  Arc_Resistance_L2L3 : powerlib/Elements/Variable Resistor  Rabsmin=1e-6
  Arc_Voltage_L1L2 : powerlib/Electrical Sources/Controlled Voltage Source  Initialize=on  Source_Type=AC  Amplitude=0  Phase=0  Frequency=0  Measurements=None
  Arc_Voltage_L2L3 : powerlib/Electrical Sources/Controlled Voltage Source  Initialize=on  Source_Type=AC  Amplitude=0  Phase=0  Frequency=0  Measurements=None
  Constant : Constant
  Current Measurement : powerlib/Measurements/Current Measurement  PhasorSimulation=off  OutputType=Complex  PSBequivalent=0
  Current Measurement1 : powerlib/Measurements/Current Measurement  PhasorSimulation=off  OutputType=Complex  PSBequivalent=0
  Demux : Demux  Outputs=2
  Demux1 : Demux  Outputs=2
  Mux : Mux  Inputs=2
  Mux1 : Mux  Inputs=2
  Mux2 : Mux  Inputs=2
  Voltage Measurement : powerlib/Measurements/Voltage Measurement  PhasorSimulation=off  OutputType=Complex  PSBequivalent=0
  Voltage Measurement1 : powerlib/Measurements/Voltage Measurement  PhasorSimulation=off  OutputType=Complex  PSBequivalent=0
  L1 : PMIOPort  Side=Right
  L2 : PMIOPort  Port=2  Side=Right
  L3 : PMIOPort  Port=3  Side=Right
  numberOfArcs : Outport
  i_arc_meas : Outport  Port=2
  v_arc_meas : Outport  Port=3
  wires:
  Current Measurement/1 -> Mux/1
  Mux/1 -> i_arc_meas/1
  Current Measurement1/1 -> Mux/2
  v_arc/1 -> Demux/1
  Demux/1 -> Arc_Voltage_L1L2/1
  Mux1/1 -> v_arc_meas/1
  Demux1/1 -> Arc_Resistance_L1L2/1
  Demux/2 -> Arc_Voltage_L2L3/1
  Voltage Measurement/1 -> Mux1/1
  Voltage Measurement1/1 -> Mux1/2
  Demux1/2 -> Arc_Resistance_L2L3/1
  Add/1 -> Demux1/1
  R_arc/1 -> Add/2
  R_block/1 -> Add/1
  Mux2/1 -> numberOfArcs/1
  Constant/1 -> Mux2/2, Mux2/1
  connections:
  Current Measurement/LConn1 -- L1/RConn1
  Current Measurement/RConn1 -- Arc_Resistance_L1L2/RConn1 -- Voltage Measurement/LConn1
  Voltage Measurement1/LConn2 -- Arc_Voltage_L2L3/LConn1 -- L3/RConn1
  Voltage Measurement/LConn2 -- Current Measurement1/LConn1 -- L2/RConn1 -- Arc_Voltage_L1L2/LConn1
  Current Measurement1/RConn1 -- Arc_Resistance_L2L3/RConn1 -- Voltage Measurement1/LConn1
  Arc_Voltage_L2L3/RConn1 -- Arc_Resistance_L2L3/LConn1
  Arc_Voltage_L1L2/RConn1 -- Arc_Resistance_L1L2/LConn1

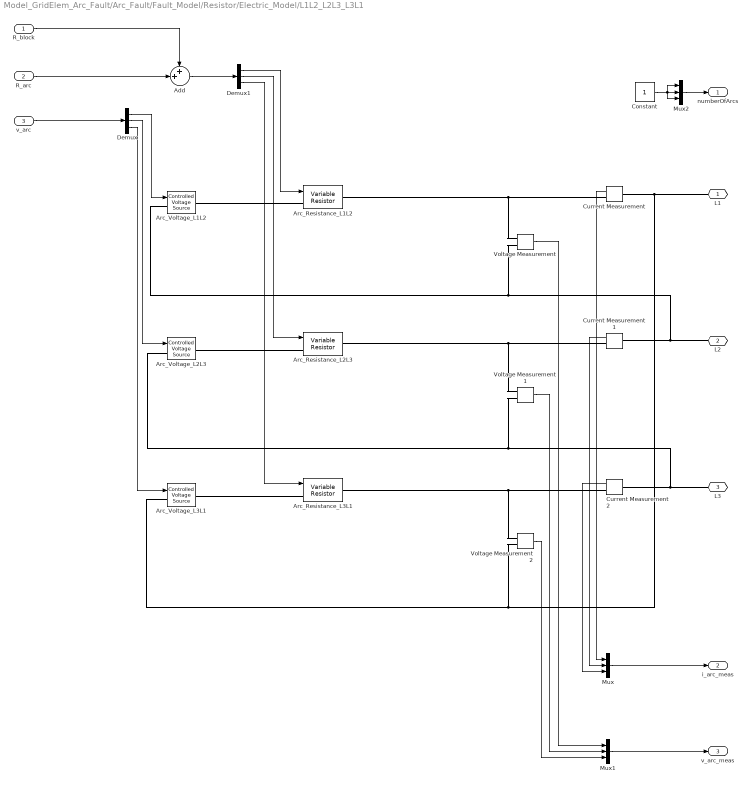
== system Model_GridElem_Arc_Fault/Arc_Fault/Fault_Model/Resistor/Electric_Model/L1L2_L2L3_L3L1 ==
  R_block : Inport
  R_arc : Inport  Port=2
  v_arc : Inport  Port=3
  Add : Sum  Inputs=++|
  Arc_Resistance_L1L2 : powerlib/Elements/Variable Resistor  Rabsmin=1e-6
  Arc_Resistance_L2L3 : powerlib/Elements/Variable Resistor  Rabsmin=1e-6
  Arc_Resistance_L3L1 : powerlib/Elements/Variable Resistor  Rabsmin=1e-6
  Arc_Voltage_L1L2 : powerlib/Electrical Sources/Controlled Voltage Source  Initialize=on  Source_Type=AC  Amplitude=0  Phase=0  Frequency=0  Measurements=None
  Arc_Voltage_L2L3 : powerlib/Electrical Sources/Controlled Voltage Source  Initialize=on  Source_Type=AC  Amplitude=0  Phase=0  Frequency=0  Measurements=None
  Arc_Voltage_L3L1 : powerlib/Electrical Sources/Controlled Voltage Source  Initialize=on  Source_Type=AC  Amplitude=0  Phase=0  Frequency=0  Measurements=None
  Constant : Constant
  Current Measurement : powerlib/Measurements/Current Measurement  PhasorSimulation=off  OutputType=Complex  PSBequivalent=0
  Current Measurement1 : powerlib/Measurements/Current Measurement  PhasorSimulation=off  OutputType=Complex  PSBequivalent=0
  Current Measurement2 : powerlib/Measurements/Current Measurement  PhasorSimulation=off  OutputType=Complex  PSBequivalent=0
  Demux : Demux  Outputs=3
  Demux1 : Demux  Outputs=3
  Mux : Mux  Inputs=3
  Mux1 : Mux  Inputs=3
  Mux2 : Mux  Inputs=3
  Voltage Measurement : powerlib/Measurements/Voltage Measurement  PhasorSimulation=off  OutputType=Complex  PSBequivalent=0
  Voltage Measurement1 : powerlib/Measurements/Voltage Measurement  PhasorSimulation=off  OutputType=Complex  PSBequivalent=0
  Voltage Measurement2 : powerlib/Measurements/Voltage Measurement  PhasorSimulation=off  OutputType=Complex  PSBequivalent=0
  L1 : PMIOPort  Side=Right
  L2 : PMIOPort  Port=2  Side=Right
  L3 : PMIOPort  Port=3  Side=Right
  numberOfArcs : Outport
  i_arc_meas : Outport  Port=2
  v_arc_meas : Outport  Port=3
  wires:
  R_block/1 -> Add/1
  Demux1/3 -> Arc_Resistance_L3L1/1
  Demux/1 -> Arc_Voltage_L1L2/1
  v_arc/1 -> Demux/1
  Demux1/1 -> Arc_Resistance_L1L2/1
  Demux/3 -> Arc_Voltage_L3L1/1
  Demux1/2 -> Arc_Resistance_L2L3/1
  Demux/2 -> Arc_Voltage_L2L3/1
  Mux/1 -> i_arc_meas/1
  Mux1/1 -> v_arc_meas/1
  Current Measurement/1 -> Mux/1
  Current Measurement1/1 -> Mux/2
  Current Measurement2/1 -> Mux/3
  Voltage Measurement/1 -> Mux1/1
  Voltage Measurement1/1 -> Mux1/2
  Voltage Measurement2/1 -> Mux1/3
  Add/1 -> Demux1/1
  R_arc/1 -> Add/2
  Mux2/1 -> numberOfArcs/1
  Constant/1 -> Mux2/3, Mux2/1, Mux2/2
  connections:
  Arc_Voltage_L1L2/RConn1 -- Arc_Resistance_L1L2/LConn1
  Arc_Voltage_L3L1/RConn1 -- Arc_Resistance_L3L1/LConn1
  Arc_Voltage_L2L3/RConn1 -- Arc_Resistance_L2L3/LConn1
  Arc_Voltage_L3L1/LConn1 -- Voltage Measurement2/LConn2 -- L1/RConn1 -- Current Measurement/LConn1
  Arc_Voltage_L2L3/LConn1 -- Voltage Measurement1/LConn2 -- Current Measurement2/LConn1 -- L3/RConn1
  L2/RConn1 -- Arc_Voltage_L1L2/LConn1 -- Voltage Measurement/LConn2 -- Current Measurement1/LConn1
  Current Measurement/RConn1 -- Arc_Resistance_L1L2/RConn1 -- Voltage Measurement/LConn1
  Current Measurement1/RConn1 -- Voltage Measurement1/LConn1 -- Arc_Resistance_L2L3/RConn1
  Current Measurement2/RConn1 -- Voltage Measurement2/LConn1 -- Arc_Resistance_L3L1/RConn1
